simulink model "Step2_Balance"  (R2026a)
settings: Solver=ode45  StopTime=8  MaxStep=0.01  RelTol=1e-8  AbsTol=1e-10
InitFcn:
  | initialise_model_visualiser(bdroot);
model workspace (MAT data in the model file):
  A_obs = [-1.03306495184  -2.62896536811  1  0; -2.62896536811  -13.6995003197  0  1; -3.98934105074  6.43487108925  -9.44823860866  -0.305475802735; -18.4818468022  -27.8933429901  -9.09170130267  -0.794477806599]
  B_obs = [0  1.03306495184  2.62896536811; 0  2.62896536811  13.6995003197; 16.9843440526  3.98934105074  20.2495570801; 16.3434254091  18.4818468022  97.2938839577]
  Bp = 0.0024
  Br = 0.0024
  C_obs = [1  0  0  0; 0  1  0  0; 0  0  1  0; 0  0  0  1]
  D_obs = [0  0  0; 0  0  0; 0  0  0; 0  0  0]
  G = 70
  J = 0.00608016405667
  Jp = 0.00119873080146
  Kx = [-3.16227766017 46.5279057069 -3.23858482369 6.80804952933]
  Lp = 0.33655
  Ra = 2.6
  alpha0 = 0.0872664625997
  disturbanceTime = 20
  disturbanceV = 0
  eta_g = 0.9
  eta_m = 0.69
  g = 9.81
  kb = 0.00768
  kt = 0.00768
  lp = 0.168275
  mp = 0.127
  r = 0.2159
  xhat0 = [0; 0; 0; 0]
values from neighbouring files (symbols this model uses):
  alphaPlotHandle = plot(inf,inf,'-b','linewidth',2)    [initialiseVisualiser.m]
  armPartPatchHandle = patch(Xt,Yt,Zt,C,'Edgecolor', edgecolor,'facealpha',facealpha,'clipping','off')    [initialiseVisualiser.m]
  armPartVertices = [X(:) Y(:) Z(:) ones(length(X(:)),1)]'    [initialiseVisualiser.m]
  drivePartPatchHandle = patch(Xt,Yt,Zt,C,'Edgecolor', edgecolor,'facealpha',facealpha,'clipping','off')    [initialiseVisualiser.m]
  drivePartVertices = [X(:) Y(:) Z(:) ones(length(X(:)),1)]'    [initialiseVisualiser.m]
  frameRate = 50    [AAP5_setup.m]
  pendPartPatchHandle = patch(Xt,Yt,Zt,C,'Edgecolor', edgecolor,'facealpha',facealpha,'clipping','off')    [initialiseVisualiser.m]
  pendPartVertices = [X(:) Y(:) Z(:) ones(length(X(:)),1)]'    [initialiseVisualiser.m]
  thetaPlotHandle = plot(inf,inf,'-r','linewidth',2)    [initialiseVisualiser.m]
settings Model: Creator=liubingnan  LastModifiedBy=DELL

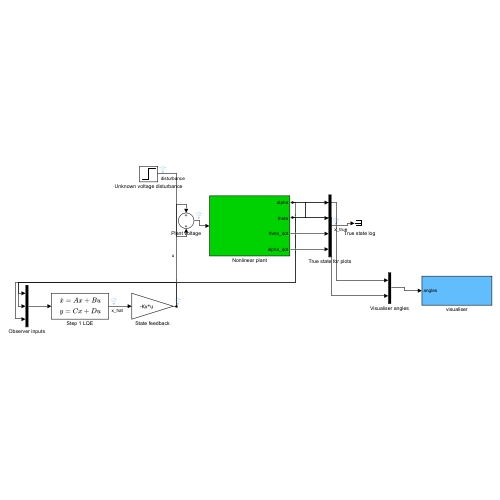
[thumbnail: Simulink's stored preview of the top-level diagram]
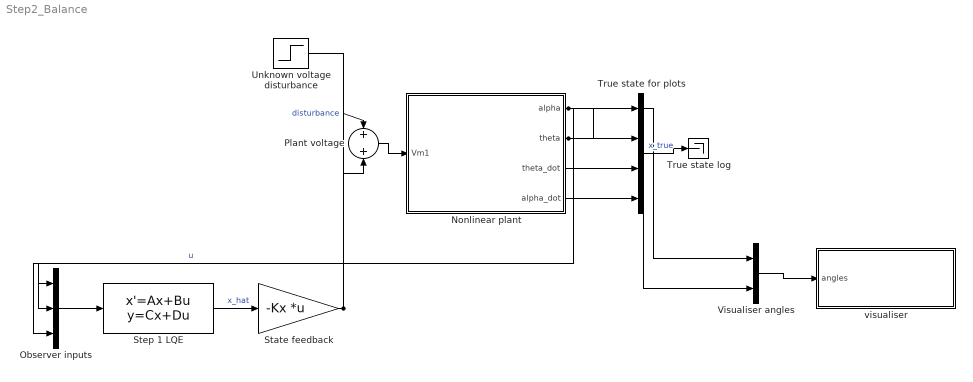
== system Step2_Balance ==
  Nonlinear plant : Subsystem
  Observer inputs : Mux  Inputs=3
  Plant voltage : Sum
  State feedback : Gain  Gain=-Kx  Multiplication=Matrix(K*u)
  Step 1 LQE : StateSpace  A=A_obs  B=B_obs  C=C_obs  D=D_obs  InitialCondition=xhat0
  True state for plots : Mux
  True state log : Terminator
  Unknown voltage disturbance : Step  Time=disturbanceTime  FinalValue=disturbanceV  SampleTime=0
  Visualiser angles : Mux  Inputs=2
  visualiser : Subsystem
  wires:
  Nonlinear plant/1(alpha) -> Visualiser angles/1, True state for plots/2, Observer inputs/3
  Nonlinear plant/2(theta) -> Visualiser angles/2, True state for plots/1, Observer inputs/2
  Visualiser angles/1 -> visualiser/1(angles)
  Unknown voltage disturbance/1 -> Plant voltage/2  "disturbance"
  Plant voltage/1 -> Nonlinear plant/1(Vm1)
  Nonlinear plant/3(theta_dot) -> True state for plots/3
  Nonlinear plant/4(alpha_dot) -> True state for plots/4
  True state for plots/1 -> True state log/1  "x_true"
  Observer inputs/1 -> Step 1 LQE/1
  Step 1 LQE/1 -> State feedback/1  "x_hat"
  State feedback/1 -> Plant voltage/1, Observer inputs/1  "u"

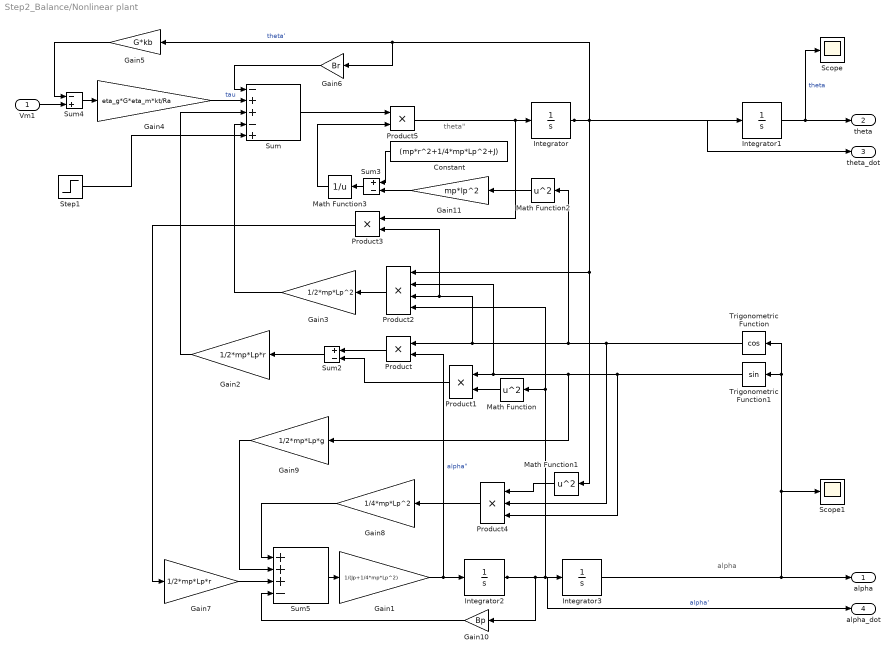
== system Step2_Balance/Nonlinear plant ==
  note: alpha
  note: theta"
  Vm1 : Inport
  Constant : Constant  Value=(mp*r^2+1/4*mp*Lp^2+J)
  Gain1 : Gain  Gain=1/(Jp+1/4*mp*Lp^2)
  Gain10 : Gain  Gain=Bp
  Gain11 : Gain  Gain=mp*lp^2
  Gain2 : Gain  Gain=1/2*mp*Lp*r
  Gain3 : Gain  Gain=1/2*mp*Lp^2
  Gain4 : Gain  Gain=eta_g*G*eta_m*kt/Ra
  Gain5 : Gain  Gain=G*kb
  Gain6 : Gain  Gain=Br
  Gain7 : Gain  Gain=1/2*mp*Lp*r
  Gain8 : Gain  Gain=1/4*mp*Lp^2
  Gain9 : Gain  Gain=1/2*mp*Lp*g
  Integrator : Integrator
  Integrator1 : Integrator
  Integrator2 : Integrator
  Integrator3 : Integrator  InitialCondition=alpha0
  Math Function : Math  Operator=square  SignedPower=on
  Math Function1 : Math  Operator=square  SignedPower=on
  Math Function2 : Math  Operator=square  SignedPower=on
  Math Function3 : Math  Operator=reciprocal  SignedPower=on
  Product{,1,3,5} (4 alike) : Product  RndMeth=Zero
  Product2 : Product  Inputs=4  RndMeth=Zero
  Product4 : Product  Inputs=3  RndMeth=Zero
  Scope : Scope
      settings: ActiveDisplayYMinimum=-1  ActiveDisplayYMaximum=1  DataLoggingVariableName=ScopeData3
  Scope1 : Scope
      settings: ActiveDisplayYMinimum=-0.00537  ActiveDisplayYMaximum=0.0023  DataLoggingVariableName=ScopeData4
  Step1 : Step  Time=.1  FinalValue=0  SampleTime=0
  Sum : Sum  Inputs=-++-+
  Sum2 : Sum  Inputs=+-
  Sum3 : Sum  Inputs=+-
  Sum4 : Sum  Inputs=-+
  Sum5 : Sum  Inputs=+++-
  Trigonometric Function : Trigonometry  Operator=cos
  Trigonometric Function1 : Trigonometry
  alpha : Outport  VectorParamsAs1DForOutWhenUnconnected=off
  theta : Outport  Port=2  VectorParamsAs1DForOutWhenUnconnected=off
  theta_dot : Outport  Port=3
  alpha_dot : Outport  Port=4
  wires:
  Integrator3/1 -> alpha/1, Trigonometric Function1/1, Trigonometric Function/1, Scope1/1
  Step1/1 -> Sum/5
  Integrator1/1 -> Scope/1, theta/1  "theta"
  Integrator/1 -> Gain5/1, Gain6/1, Integrator1/1, Product2/1, Math Function1/1, theta_dot/1  "theta'"
  Trigonometric Function/1 -> Math Function2/1, Product/1, Product2/3, Product3/2, Product4/2
  Gain1/1 -> Integrator2/1, Product/2  "alpha\""
  Integrator2/1 -> Product2/4, Math Function/1, Integrator3/1, Gain10/1, alpha_dot/1  "alpha'"
  Math Function1/1 -> Product4/1
  Gain8/1 -> Sum5/1
  Gain3/1 -> Sum/4
  Gain6/1 -> Sum/1
  Gain4/1 -> Sum/2  "tau"
  Sum4/1 -> Gain4/1
  Gain5/1 -> Sum4/1
  Vm1/1 -> Sum4/2
  Product2/1 -> Gain3/1
  Product4/1 -> Gain8/1
  Product1/1 -> Sum2/2
  Math Function/1 -> Product1/2
  Trigonometric Function1/1 -> Product1/1, Product2/2, Gain9/1, Product4/3
  Product3/1 -> Gain7/1
  Gain7/1 -> Sum5/3
  Gain2/1 -> Sum/3
  Sum5/1 -> Gain1/1
  Math Function3/1 -> Product5/2
  Sum3/1 -> Math Function3/1
  Constant/1 -> Sum3/1
  Gain11/1 -> Sum3/2
  Math Function2/1 -> Gain11/1
  Gain10/1 -> Sum5/4
  Gain9/1 -> Sum5/2
  Sum/1 -> Product5/1
  Sum2/1 -> Gain2/1
  Product/1 -> Sum2/1
  Product5/1 -> Integrator/1, Product3/1

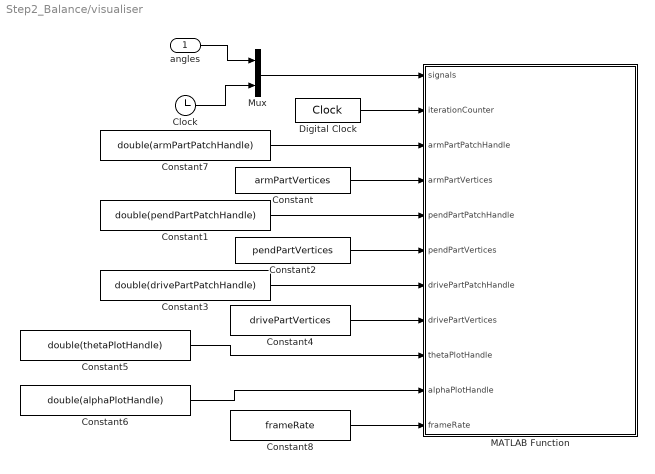
== system Step2_Balance/visualiser ==
  angles : Inport
  Clock : Clock
  Constant : Constant  Value=armPartVertices  VectorParams1D=off
  Constant1 : Constant  Value=double(pendPartPatchHandle)
  Constant2 : Constant  Value=pendPartVertices  VectorParams1D=off
  Constant3 : Constant  Value=double(drivePartPatchHandle)
  Constant4 : Constant  Value=drivePartVertices  VectorParams1D=off
  Constant5 : Constant  Value=double(thetaPlotHandle)
  Constant6 : Constant  Value=double(alphaPlotHandle)
  Constant7 : Constant  Value=double(armPartPatchHandle)
  Constant8 : Constant  Value=frameRate  VectorParams1D=off
  Digital Clock : DigitalClock  SampleTime=.001
  MATLAB Function : MATLAB Function  TreatAsAtomicUnit=on
  Mux : Mux  Inputs=2
  wires:
  Constant8/1 -> MATLAB Function/11(frameRate)
  Digital Clock/1 -> MATLAB Function/2(iterationCounter)
  Constant3/1 -> MATLAB Function/7(drivePartPatchHandle)
  Constant4/1 -> MATLAB Function/8(drivePartVertices)
  Constant5/1 -> MATLAB Function/9(thetaPlotHandle)
  Constant6/1 -> MATLAB Function/10(alphaPlotHandle)
  Constant2/1 -> MATLAB Function/6(pendPartVertices)
  Constant1/1 -> MATLAB Function/5(pendPartPatchHandle)
  Constant/1 -> MATLAB Function/4(armPartVertices)
  Constant7/1 -> MATLAB Function/3(armPartPatchHandle)
  Clock/1 -> Mux/2
  Mux/1 -> MATLAB Function/1(signals)
  angles/1 -> Mux/1

== matlab function Step2_Balance/visualiser/MATLAB Function ==
  data: signals input; iterationCounter input; armPartPatchHandle input; armPartVertices input; pendPartPatchHandle input; pendPartVertices input; drivePartPatchHandle input; drivePartVertices input; thetaPlotHandle input; alphaPlotHandle input; frameRate input
function  updateVisualiser(signals, iterationCounter, armPartPatchHandle, armPartVertices, pendPartPatchHandle, pendPartVertices, drivePartPatchHandle, drivePartVertices, thetaPlotHandle, alphaPlotHandle, frameRate)

%
% We need the set and get functions for changing plots.
%
coder.extrinsic('set');
coder.extrinsic('get');


%
% Clear the theta and alpha plots if this is the first iteration.
%
if iterationCounter == 0
    set(thetaPlotHandle,'xData',inf,'yData',inf);
    set(alphaPlotHandle,'xData',inf,'yData',inf);
end

%
% Only update figure on every 2nd iteration.
%
if mod(iterationCounter,1/frameRate) == 0
    
    alphaAngle = signals(1);
    thetaAngle = signals(2);
    currentTime = signals(3);
    
    %
    % New frame transformations.
    %
    BaseToArm = homogeneous_func(0,0,thetaAngle,0,0,12e-2);
    ArmToPendulum = homogeneous_func(alphaAngle,0,0,14.2e-2,0,5e-2);
    BaseToDrive = homogeneous_func(0,0,(-thetaAngle*5),0,0.036,12e-2);
    
    %
    % Update arm parts.
    %
    armPart_vertices_G_frame = BaseToArm * armPartVertices;
    Xt = reshape(armPart_vertices_G_frame(1,:),3,[]);
    Yt = reshape(armPart_vertices_G_frame(2,:),3,[]);
    Zt = reshape(armPart_vertices_G_frame(3,:),3,[]);
    set(armPartPatchHandle, 'xData', Xt, 'yData', Yt, 'zData', Zt);
    
    %
    % Update pendulum parts.
    %
    pendPart_vertices_G_frame = BaseToArm * ArmToPendulum* pendPartVertices;
    Xt = reshape(pendPart_vertices_G_frame(1,:),3,[]);
    Yt = reshape(pendPart_vertices_G_frame(2,:),3,[]);
    Zt = reshape(pendPart_vertices_G_frame(3,:),3,[]);
    set(pendPartPatchHandle, 'xData', Xt, 'yData', Yt, 'zData', Zt);
    
    %
    % Update drive gear parts.
    %
    drivePart_vertices_G_frame = BaseToDrive* drivePartVertices;
    Xt = reshape(drivePart_vertices_G_frame(1,:),3,[]);
    Yt = reshape(drivePart_vertices_G_frame(2,:),3,[]);
    Zt = reshape(drivePart_vertices_G_frame(3,:),3,[]);
    set(drivePartPatchHandle, 'xData', Xt, 'yData', Yt, 'zData', Zt);
    
    %
    % Update theta plot.
    %
    times = [get(thetaPlotHandle,'xData'), currentTime];
    thetaAngles = [get(thetaPlotHandle,'yData'), thetaAngle*180/pi];
    set(thetaPlotHandle,'xdata',times,'ydata',thetaAngles);
    
    %
    % Update alpha plot.
    %
    times = [get(alphaPlotHandle,'xData'), currentTime];
    alphaAngles = [get(alphaPlotHandle,'yData'), alphaAngle*180/pi];
    set(alphaPlotHandle,'xdata',times,'ydata',alphaAngles);
end
end

function [T] = homogeneous_func(ROLL, PITCH, YAW, X, Y, Z)
T=zeros(4,4);
T(1,1) = cos(YAW)*cos(PITCH);
T(1,2) = cos(YAW)*sin(PITCH)*sin(ROLL)-sin(YAW)*cos(ROLL);
T(1,3) = cos(YAW)*sin(PITCH)*cos(ROLL)+sin(YAW)*sin(ROLL);
T(1,4) = X;
T(2,1) = sin(YAW)*cos(PITCH);
T(2,2) = sin(YAW)*sin(PITCH)*sin(ROLL)+cos(YAW)*cos(ROLL);
T(2,3) = sin(YAW)*sin(PITCH)*cos(ROLL)-cos(YAW)*sin(ROLL);
T(2,4) = Y;
T(3,1) = -sin(PITCH);
T(3,2) = cos(PITCH)*sin(ROLL);
T(3,3) = cos(PITCH)*cos(ROLL);
T(3,4) = Z;
T(4,4) = 1;
end
